simulink model "RTR"  (R2023b)
settings: Solver=VariableStepAuto  StartTime=0.0  StopTime=10.0  RelTol=1e-3
settings Model: Creator=user  LastModifiedBy=user

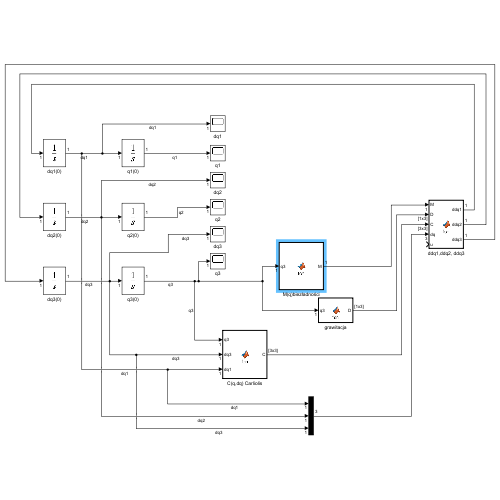
[thumbnail: Simulink's stored preview of the top-level diagram]
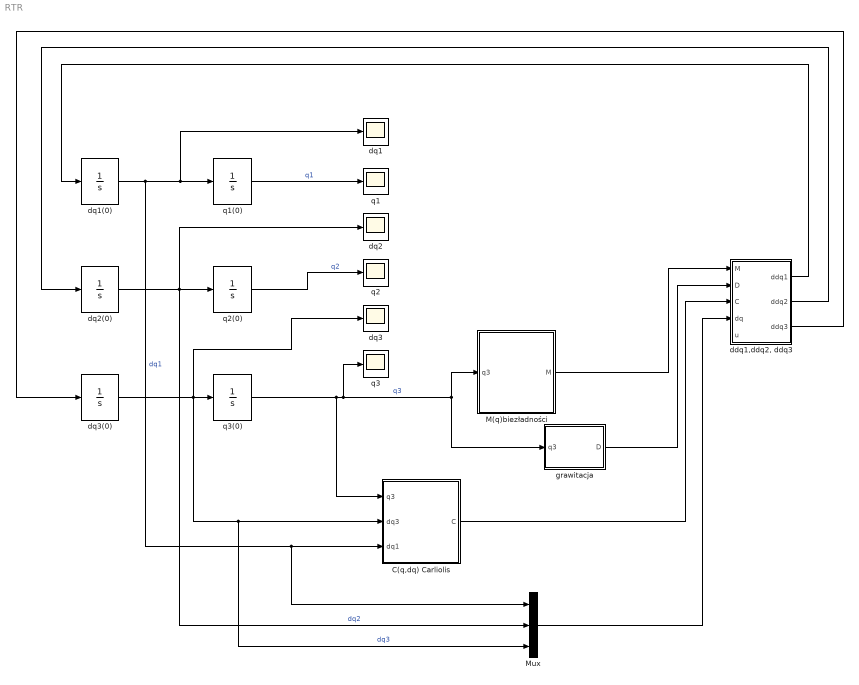
== system RTR ==
  C(q,dq) Carliolis : MATLAB Function  TreatAsAtomicUnit=on
  M(q)biezładności : MATLAB Function  TreatAsAtomicUnit=on
  Mux : Mux  Inputs=3
  "ddq1,ddq2, ddq3" : MATLAB Function  TreatAsAtomicUnit=on
  dq1 : Scope
  dq1(0) : Integrator
  dq2 : Scope
  dq2(0) : Integrator
  dq3 : Scope
  dq3(0) : Integrator
  grawitacja : MATLAB Function  TreatAsAtomicUnit=on
  q1 : Scope
  q1(0) : Integrator
  q2 : Scope
  q2(0) : Integrator
  q3 : Scope
  q3(0) : Integrator
  wires:
  dq1(0)/1 -> dq1/1, q1(0)/1, Mux/1, C(q,dq) Carliolis/3(dq1)  "dq1"
  q1(0)/1 -> q1/1  "q1"
  q2(0)/1 -> q2/1  "q2"
  dq2(0)/1 -> Mux/2, dq2/1, q2(0)/1  "dq2"
  q3(0)/1 -> C(q,dq) Carliolis/1(q3), grawitacja/1(q3), M(q)biezładności/1(q3), q3/1  "q3"
  dq3(0)/1 -> dq3/1, Mux/3, C(q,dq) Carliolis/2(dq3), q3(0)/1  "dq3"
  C(q,dq) Carliolis/1(C) -> "ddq1,ddq2, ddq3"/3(C)
  M(q)biezładności/1(M) -> "ddq1,ddq2, ddq3"/1(M)
  grawitacja/1(D) -> "ddq1,ddq2, ddq3"/2(D)
  Mux/1 -> "ddq1,ddq2, ddq3"/4(dq)
  "ddq1,ddq2, ddq3"/1(ddq1) -> dq1(0)/1
  "ddq1,ddq2, ddq3"/2(ddq2) -> dq2(0)/1
  "ddq1,ddq2, ddq3"/3(ddq3) -> dq3(0)/1

== matlab function RTR/C(q,dq) Carliolis ==
  data: q3 input; dq3 input; dq1 input; C output
function C  = fcn(q3, dq3, dq1)

I = (0.6 * sin(q3) + 0.2667 * sin(q3) *cos(q3));

C11 = -dq3 * I;
C12 = 0;
C31 = dq1 * I;
C13 = -dq1 * I;
C23 = -dq3 * 0.6 * sin(q3);

C = [C11, 0, C13;
      0,  0, C23;
     C31, 0,  0];


end

== matlab function RTR/M(q)biezładności ==
  data: q3 input; M output
function M  = fcn(q3)

M12 = 0;
M23 = 0.6 * cos(q3);

M11 = 2.4 + 0.2667 * cos(q3) + 1.2 * cos(q3);
M22 = 40;
M33 = 0.2667;

 M = [M11,   0,      0;
        0, M22,    M23;
        0, M23, 0.2667 ];
 
end

== matlab function RTR/grawitacja ==
  data: q3 input; D output
function  D = fcn(q3)

D1 = 0;
D2 = 362;
D3 = 19.6 * sin(q3);
D = [D1,D2,D3];

end

== matlab function RTR/ddq1,ddq2, ddq3 ==
  data: M input; D input; C input; dq input; u input; ddq1 output; ddq2 output; ddq3 output
function [ddq1, ddq2, ddq3] = fcn(M, D, C, dq, u)

ddq = M \ (u - C * dq - D);

ddq1 = ddq(1);
ddq2 = ddq(2);
ddq3 = ddq(3);

end
